simulink model "GameBoard_Fall26"  (R2026a)
settings: Solver=FixedStepAuto  StopTime=inf  FixedStep=0.001  EnableMultiTasking=on
model workspace (MAT data in the model file):
  Error = 0
libraries: arduinolib x5, slpidlib x1
settings Model: SimulationMode=external  SILPILModeSetting=veronly  ExtModeTrigDuration=2  Creator=Ninad  LastModifiedBy=ejarr
settings DataIOCC: SignalLoggingSaveFormat=ModelDataLogs  LoggingToFile=on
settings OptimizationCC: PassReuseOutputArgsThreshold=0.0
settings DebuggingCC: UnderspecifiedInitializationDetection=Classic  MultiTaskRateTransMsg=warning
settings HardwareCC: ProdBitPerInt=16.0  ProdBitPerPointer=16.0  ProdBitPerSizeT=16.0  ProdBitPerPtrDiffT=16.0  ProdWordSize=8.0  ProdHWDeviceType=Atmel->AVR  UseEmbeddedCoderFeatures=off
settings RTWCC: SystemTargetFile=ert.tlc  HardwareBoard=Arduino Mega 2560  TLCOptions=-aInlineSetEventsForThisBaseRateFcn=TLC_FALSE -aSuppressMultiTaskScheduler=TLC_FALSE -aRateBasedStepFcn=1  Toolchain=Arduino AVR  BuildConfiguration=Faster Runs  Description=Embedded Coder
settings ERTTargetCC: ExtMode=on  ExtModeStaticAllocSize=2048.0  ExtModeMexArgs='' 1 17725  ERTSrcFileBannerTemplate=codertarget_code_template.cgt  ERTHdrFileBannerTemplate=codertarget_code_template.cgt  ERTDataSrcFileTemplate=codertarget_code_template.cgt  ERTDataHdrFileTemplate=codertarget_code_template.cgt  DynamicArrayContainerType=coder::array  CodeReplacementLibrary=GNU C99 extensions  ERTCustomFileBanners=off  SupportContinuousTime=on  SupportNonInlinedSFcns=on  SupportVariableSizeSignals=on  ModelStepFunctionPrototypeControlCompliant=off

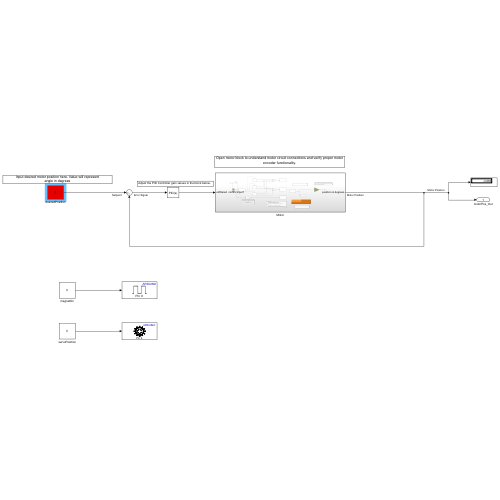
[thumbnail: Simulink's stored preview of the top-level diagram]
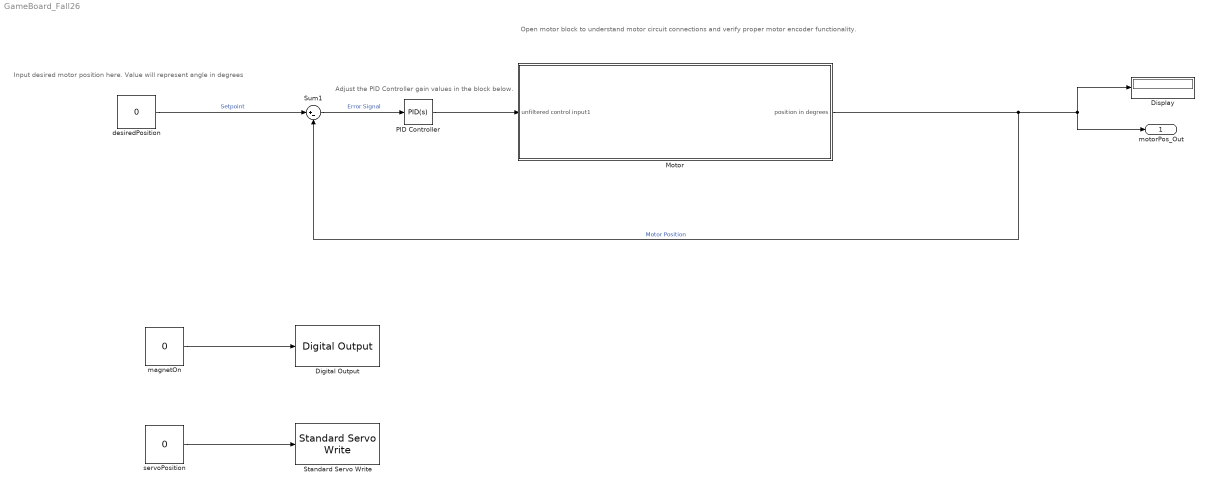
== system GameBoard_Fall26 ==
  note: Adjust the PID Controller gain values in the block below.
  note: Input desired motor position here. Value will represent
      | angle in degrees
  note: Open motor block to understand motor circuit connections and verify proper motor encoder functionality.
  Digital Output : arduinolib/Digital Output  pinNumber=8  Direction=output  blockPlatform=arduino
  Display : Display
  Motor : Subsystem
  PID Controller : slpidlib/PID Controller  Controller=PID  Form=Parallel  TimeDomain=Continuous-time  UseExternalTs=off  SampleTime=-1  IntegratorMethod=Forward Euler  FilterMethod=Forward Euler  ControllerParametersSource=internal  P=.8  I=0  UseKiTs=off  D=.05  UseExternalDerivativeSource=off  N=200  UseFilter=on  TunerSelectOption=Transfer Function Based (PID Tuner App)  InitialConditionSource=internal  InitialConditionForIntegrator=0  InitialConditionForFilter=0  DifferentiatorICPrevScaledInput=0  ExternalReset=none  TrackingMode=off  Kt=1  LimitOutput=off  SatLimitsSource=internal  UpperSaturationLimit=inf  LowerSaturationLimit=-inf  LinearizeAsGain=on  AntiWindupMode=none  Kb=1  LimitIntegrator=off  UpperIntegratorSaturationLimit=inf  LowerIntegratorSaturationLimit=-inf  POutMin=[]  POutMax=[]  IOutMin=[]  IOutMax=[]  DOutMin=[]  DOutMax=[]  NOutMin=[]  NOutMax=[]  SumOutMin=[]  SumOutMax=[]  SaturationOutMin=[]  SaturationOutMax=[]  PParamMin=[]  PParamMax=[]  IParamMin=[]  IParamMax=[]  DParamMin=[]  DParamMax=[]  NParamMin=[]  NParamMax=[]  KbParamMin=[]  KbParamMax=[]  KtParamMin=[]  KtParamMax=[]  KbOutMin=[]  KbOutMax=[]  KtOutMin=[]  KtOutMax=[]  IntegratorOutMin=[]  IntegratorOutMax=[]  FilterOutMin=[]  FilterOutMax=[]  SumI1OutMin=[]  SumI1OutMax=[]  SumI2OutMin=[]  SumI2OutMax=[]  SumI3OutMin=[]  SumI3OutMax=[]  SumI4OutMin=[]  SumI4OutMax=[]  SumDOutMin=[]  SumDOutMax=[]  DifferentiatorOutMin=[]  DifferentiatorOutMax=[]  FilterDiffOutCoefMin=[]  FilterDiffOutCoefMax=[]  ReciprocalOutMin=[]  ReciprocalOutMax=[]  SumDenOutMin=[]  SumDenOutMax=[]  SumNumOutMin=[]  SumNumOutMax=[]  DivideOutMin=[]  DivideOutMax=[]  UdiffTsProdOutMin=[]  UdiffTsProdOutMax=[]  NTsProdOutMin=[]  NTsProdOutMax=[]  UintegralTsProdOutMin=[]  UintegralTsProdOutMax=[]  UngainTsProdOutMin=[]  UngainTsProdOutMax=[]  ClampingZeroOutDataTypeStr=Inherit: Inherit via back propagation  ClampingZeroOutMin=[]  ClampingZeroOutMax=[]  FilterDenConstantOutDataTypeStr=Inherit: Inherit via back propagation  FilterDenConstantOutMin=[]  FilterDenConstantOutMax=[]  PCopyOutDataTypeStr=Inherit: Inherit via back propagation  PCopyOutMin=[]  PCopyOutMax=[]  NCopyOutDataTypeStr=Inherit: Inherit via back propagation  NCopyOutMin=[]  NCopyOutMax=[]  IntegratorContinuousStateAttributes=''  IntegratorStateMustResolveToSignalObject=off  IntegratorRTWStateStorageClass=Auto  FilterContinuousStateAttributes=''  FilterStateMustResolveToSignalObject=off  FilterRTWStateStorageClass=Auto  ParallelPVariant=InternalParameters  IdealPVariant=Disabled  IVariant=InternalParameters  DVariant=InternalParameters  IntegratorVariant=Continuous  SatVariant=Disabled  AWVariant=Passthrough  PCopyVariant=Disabled  TRVariant=Disabled  FdbkBlocksVariant=Forward  IdealPFdbkVariant=Disabled  SatFdbkVariant=Disabled  DerivativeFilterVariant=ContFilter  NVariant=InternalParameters  NCopyVariant=Disabled  FilterICVariant=InternalICsFilter  IntegratorICVariant=InternalICs  ExternalResetVariant=Disabled  TRSumVariant=Passthrough  SumFdbkVariant=Disabled  SumVariant=Sum_PID  TsampFilterVariant=InternalTs  TsampNgainVariant=Passthrough  TsampIntegralVariant=Disabled_SignalSpec  ExternalSaturationOutDataTypeStr=Inherit: Same as second input  DerivativeSourceVariant=ErrorSignal  PreIntVariant=InternalPreInt
  Standard Servo Write : arduinolib/Standard Servo Write  pinNumber=9  ServoIndex=0  blockPlatform=ARDUINO
  Sum1 : Sum  Inputs=|+-
  desiredPosition : Constant  Value=0
  magnetOn : Constant  Value=0
  servoPosition : Constant  Value=0
  motorPos_Out : Outport  VectorParamsAs1DForOutWhenUnconnected=off
  wires:
  desiredPosition/1 -> Sum1/1  "Setpoint"
  Motor/1(position in degrees) -> motorPos_Out/1, Display/1, Sum1/2  "Motor Position"
  Sum1/1 -> PID Controller/1  "Error Signal"
  PID Controller/1 -> Motor/1(unfiltered control input1)
  servoPosition/1 -> Standard Servo Write/1
  magnetOn/1 -> Digital Output/1

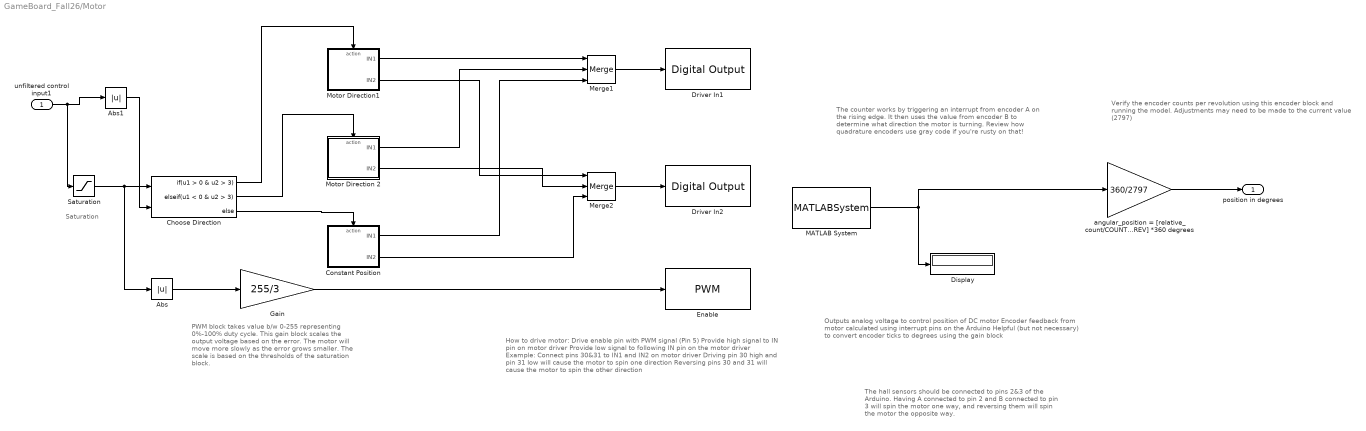
== system GameBoard_Fall26/Motor ==
  note: The counter works by triggering an interrupt from encoder A
      | on the rising edge. It then uses the value from encoder B to
      | determine what direction the motor is turning. Review how
      | quadrature encoders use gray code if you're rusty on that!
  note: PWM block takes value b/w 0-255 representing
      | 0%-100% duty cycle. This gain block scales the
      | output voltage based on the error. The motor will
      | move more slowly as the error grows
      | smaller. The scale is based on the thresholds
      | of the saturation block.
  note: Outputs analog voltage to control position of DC motor
      |
      | Encoder feedback from motor calculated using interrupt pins on the Arduino
      |
      | Helpful (but not necessary) to convert encoder ticks to degrees using the
      | gain block
  note: Saturation
  note: How to drive motor:
      | Drive enable pin with PWM signal (Pin 5)
      | Provide high signal to IN pin on motor driver
      | Provide low signal to following IN pin on the motor driver
      |
      | Example:
      | Connect pins 30&31 to IN1 and IN2 on motor driver
      | Driving pin 30 high and pin 31 low will cause the motor to spin one direction
      | Reversing pins 30 and 31 will cause the motor to spin the other direction
  note: The hall sensors should be connected to pins 2&3 of the
      | Arduino. Having A connected to pin 2 and B connected to
      | pin 3 will spin the motor one way, and reversing them will
      | spin the motor the opposite way.
  note: Verify the encoder counts per revolution using this encoder
      | block and running the model. Adjustments may need to be
      | made to the current value (2797)
  unfiltered control input1 : Inport
  Abs : Abs  SaturateOnIntegerOverflow=off
  Abs1 : Abs  SaturateOnIntegerOverflow=off
  Choose Direction : If  NumInputs=2  IfExpression=u1 > 0 & u2 > 3  ElseIfExpressions=u1 < 0 & u2 > 3
  Constant Position : Subsystem  TreatAsAtomicUnit=on
  Display : Display
  Driver In1 : arduinolib/Digital Output  pinNumber=30  Direction=output  blockPlatform=arduino
  Driver In2 : arduinolib/Digital Output  pinNumber=31  Direction=output  blockPlatform=arduino
  Enable : arduinolib/PWM  pinNumber=5  frequencyType=Default  desiredFrequency=490.2  achievableFrequency=490.2
  Gain : Gain  Gain=255/3
  MATLAB System : MATLABSystem  System=Encoder_arduino  Encoder=0  PinA=2  PinB=3  SampleTime=0.001
      mask Type: Encoder_arduino
  Merge1 : Merge  Inputs=3
  Merge2 : Merge  Inputs=3
  Motor Direction 2 : Subsystem  TreatAsAtomicUnit=on
  Motor Direction1 : Subsystem  TreatAsAtomicUnit=on
  Saturation : Saturate  UpperLimit=5  LowerLimit=-5
  angular_position = [relative_count/COUNTS_PER_REV] *360 degrees : Gain  Gain=360/2797
  position in degrees : Outport  VectorParamsAs1DForOutWhenUnconnected=off
  wires:
  angular_position = [relative_count/COUNTS_PER_REV] *360 degrees/1 -> position in degrees/1
  Saturation/1 -> Abs/1, Choose Direction/1
  Choose Direction/1 -> Motor Direction1/Action
  Motor Direction1/1(IN1) -> Merge1/1
  Motor Direction 2/1(IN1) -> Merge1/2
  Motor Direction1/2(IN2) -> Merge2/1
  Motor Direction 2/2(IN2) -> Merge2/2
  Abs/1 -> Gain/1
  Gain/1 -> Enable/1
  Merge1/1 -> Driver In1/1
  Merge2/1 -> Driver In2/1
  Constant Position/2(IN2) -> Merge2/3
  Constant Position/1(IN1) -> Merge1/3
  unfiltered control input1/1 -> Saturation/1, Abs1/1
  Abs1/1 -> Choose Direction/2
  Choose Direction/3 -> Constant Position/Action
  Choose Direction/2 -> Motor Direction 2/Action
  MATLAB System/1 -> Display/1, angular_position = [relative_count/COUNTS_PER_REV] *360 degrees/1

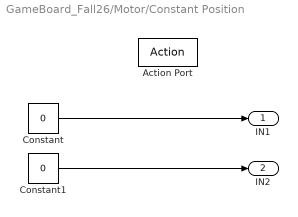
== system GameBoard_Fall26/Motor/Constant Position ==
  Action Port : ActionPort  ActionPortLabel=else
  Constant : Constant  Value=0
  Constant1 : Constant  Value=0
  IN1 : Outport
  IN2 : Outport  Port=2
  wires:
  Constant/1 -> IN1/1
  Constant1/1 -> IN2/1

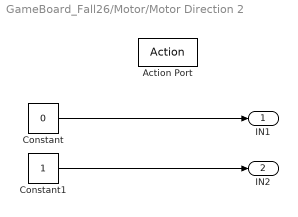
== system GameBoard_Fall26/Motor/Motor Direction 2 ==
  Action Port : ActionPort  ActionPortLabel=elseif(u1 < 0 & u2 > 3)
  Constant : Constant  Value=0
  Constant1 : Constant
  IN1 : Outport
  IN2 : Outport  Port=2
  wires:
  Constant/1 -> IN1/1
  Constant1/1 -> IN2/1

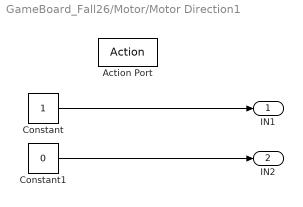
== system GameBoard_Fall26/Motor/Motor Direction1 ==
  Action Port : ActionPort  ActionPortLabel=if(u1 > 0 & u2 > 3)
  Constant : Constant
  Constant1 : Constant  Value=0
  IN1 : Outport
  IN2 : Outport  Port=2
  wires:
  Constant/1 -> IN1/1
  Constant1/1 -> IN2/1
